simulink model "quadrotor_1d"  (R2025b)
settings: Solver=VariableStepAuto  StartTime=0.0  StopTime=20  RelTol=1e-3
values from neighbouring files (symbols this model uses):
  c_d = 0.1    [quad_params.m]
  g = 9.81    [quad_params.m]
  k_f = m*g/(4*w_hover^2)    (= 5.00510204082e-06)    [quad_params.m]
  Kd = m*(2*zeta*wn + alpha)    [design_pid.m]
  Ki = m*(alpha*wn^2)    [design_pid.m]
  Kp = m*(wn^2 + 2*zeta*wn*alpha)    [design_pid.m]
  m = 1.0    (= 1)    [quad_params.m]
  tau_m = 0.05    [quad_params.m]
  U_max = 2*m*g    (= 19.62)    [quad_params.m]
  w_hover = 700    [quad_params.m]
  w_max = sqrt(U_max/(4*k_f))    [quad_params.m]
  wind_amp = -6    [quad_params.m]
  wind_dur = 3    [quad_params.m]
  wind_t0 = 5    [quad_params.m]
  z0 = 0    [quad_params.m]
settings Model: Creator=Monster  LastModifiedBy=Monster

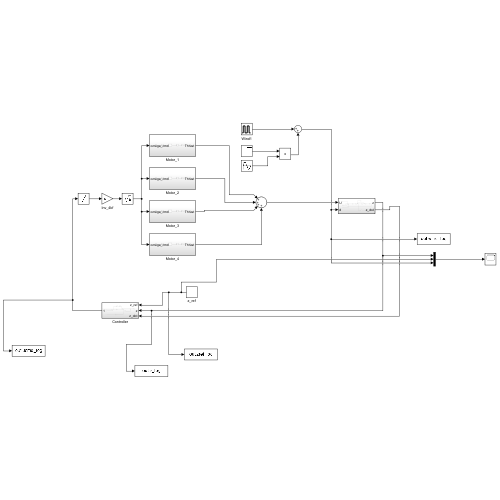
[thumbnail: Simulink's stored preview of the top-level diagram]
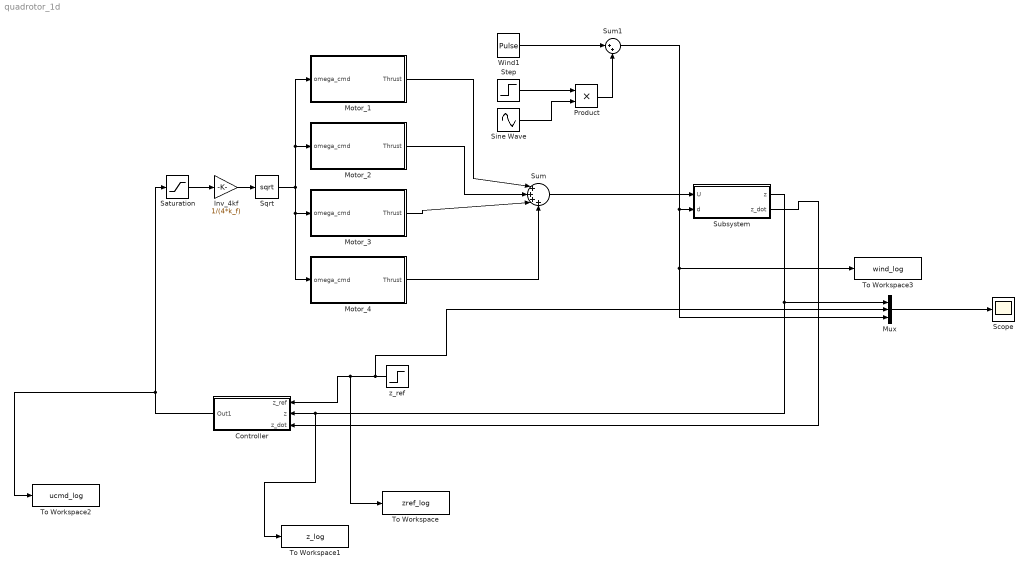
== system quadrotor_1d ==
  Controller : Subsystem
  Inv_4kf : Gain  Gain=1/(4*k_f)
  Motor_1 : Subsystem
  Motor_2 : Subsystem
  Motor_3 : Subsystem
  Motor_4 : Subsystem
  Mux : Mux  Inputs=3
  Product : Product
  Saturation : Saturate  UpperLimit=U_max  LowerLimit=0
  Scope : Scope
      settings: ActiveDisplayYMinimum=-11.330608642093068  ActiveDisplayYMaximum=2.393195803335681
  Sine Wave : Sin  Amplitude=3  Frequency=2  Phase=-24  SampleTime=0
  Sqrt : Sqrt
  Step : Step  Time=12  SampleTime=0
  Subsystem : Subsystem
  Sum : Sum  Inputs=|++++
  Sum1 : Sum  Inputs=|++
  To Workspace : ToWorkspace  VariableName=zref_log  SampleTime=-1
  To Workspace1 : ToWorkspace  VariableName=z_log  SampleTime=-1
  To Workspace2 : ToWorkspace  VariableName=ucmd_log  SampleTime=-1
  To Workspace3 : ToWorkspace  VariableName=wind_log  SampleTime=-1
  Wind1 : DiscretePulseGenerator  PulseType=Time based  Amplitude=wind_amp  Period=20  PulseWidth=100*wind_dur/20  PhaseDelay=wind_t0
  z_ref : Step  After=0.2  SampleTime=0
  wires:
  Inv_4kf/1 -> Sqrt/1
  Controller/1(Out1) -> To Workspace2/1, Saturation/1
  Saturation/1 -> Inv_4kf/1
  Sqrt/1 -> Motor_2/1(omega_cmd), Motor_1/1(omega_cmd), Motor_4/1(omega_cmd), Motor_3/1(omega_cmd)
  Motor_1/1(Thrust) -> Sum/1
  Motor_2/1(Thrust) -> Sum/2
  Motor_3/1(Thrust) -> Sum/3
  Motor_4/1(Thrust) -> Sum/4
  Sum/1 -> Subsystem/1(U)
  Sum1/1 -> Mux/3, To Workspace3/1, Subsystem/2(d)
  Subsystem/2(z_dot) -> Controller/3(z_dot)
  Subsystem/1(z) -> To Workspace1/1, Controller/2(z), Mux/1
  Mux/1 -> Scope/1
  z_ref/1 -> Mux/2, To Workspace/1, Controller/1(z_ref)
  Sine Wave/1 -> Product/2
  Step/1 -> Product/1
  Wind1/1 -> Sum1/1
  Product/1 -> Sum1/2

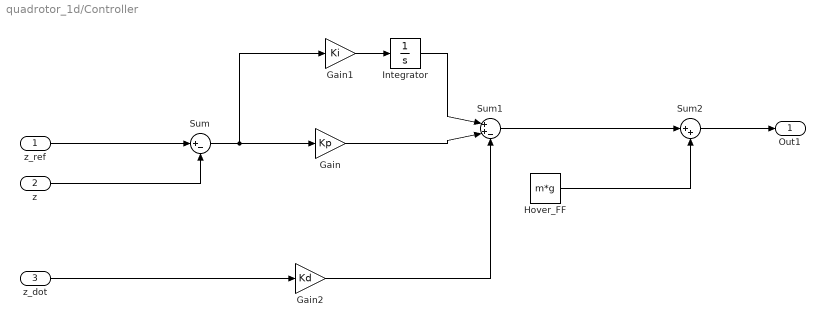
== system quadrotor_1d/Controller ==
  z_ref : Inport
  z : Inport  Port=2
  z_dot : Inport  Port=3
  Gain : Gain  Gain=Kp
  Gain1 : Gain  Gain=Ki
  Gain2 : Gain  Gain=Kd
  Hover_FF : Constant  Value=m*g
  Integrator : Integrator
  Sum : Sum  Inputs=|+-
  Sum1 : Sum  Inputs=|++-
  Sum2 : Sum  Inputs=|++
  Out1 : Outport
  wires:
  z_ref/1 -> Sum/1
  z/1 -> Sum/2
  Sum/1 -> Gain1/1, Gain/1
  Gain1/1 -> Integrator/1
  Integrator/1 -> Sum1/1
  Gain/1 -> Sum1/2
  z_dot/1 -> Gain2/1
  Gain2/1 -> Sum1/3
  Sum1/1 -> Sum2/1
  Hover_FF/1 -> Sum2/2
  Sum2/1 -> Out1/1

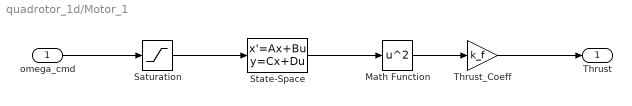
== system quadrotor_1d/Motor_1 ==
  omega_cmd : Inport
  Math Function : Math  Operator=square
  Saturation : Saturate  UpperLimit=w_max  LowerLimit=0
  State-Space : StateSpace  A=-1/tau_m  B=1/tau_m  D=0  InitialCondition=w_hover
  Thrust_Coeff : Gain  Gain=k_f
  Thrust : Outport
  wires:
  Thrust_Coeff/1 -> Thrust/1
  Saturation/1 -> State-Space/1
  State-Space/1 -> Math Function/1
  Math Function/1 -> Thrust_Coeff/1
  omega_cmd/1 -> Saturation/1

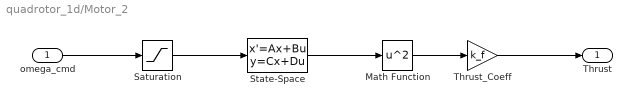
== system quadrotor_1d/Motor_2 ==
  omega_cmd : Inport
  Math Function : Math  Operator=square
  Saturation : Saturate  UpperLimit=w_max  LowerLimit=0
  State-Space : StateSpace  A=-1/tau_m  B=1/tau_m  D=0  InitialCondition=w_hover
  Thrust_Coeff : Gain  Gain=k_f
  Thrust : Outport
  wires:
  Thrust_Coeff/1 -> Thrust/1
  Saturation/1 -> State-Space/1
  State-Space/1 -> Math Function/1
  Math Function/1 -> Thrust_Coeff/1
  omega_cmd/1 -> Saturation/1

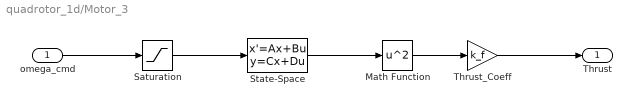
== system quadrotor_1d/Motor_3 ==
  omega_cmd : Inport
  Math Function : Math  Operator=square
  Saturation : Saturate  UpperLimit=w_max  LowerLimit=0
  State-Space : StateSpace  A=-1/tau_m  B=1/tau_m  D=0  InitialCondition=w_hover
  Thrust_Coeff : Gain  Gain=k_f
  Thrust : Outport
  wires:
  Thrust_Coeff/1 -> Thrust/1
  Saturation/1 -> State-Space/1
  State-Space/1 -> Math Function/1
  Math Function/1 -> Thrust_Coeff/1
  omega_cmd/1 -> Saturation/1

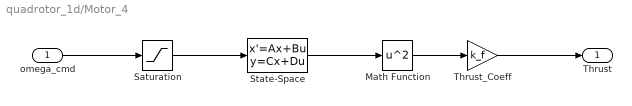
== system quadrotor_1d/Motor_4 ==
  omega_cmd : Inport
  Math Function : Math  Operator=square
  Saturation : Saturate  UpperLimit=w_max  LowerLimit=0
  State-Space : StateSpace  A=-1/tau_m  B=1/tau_m  D=0  InitialCondition=w_hover
  Thrust_Coeff : Gain  Gain=k_f
  Thrust : Outport
  wires:
  Thrust_Coeff/1 -> Thrust/1
  Saturation/1 -> State-Space/1
  State-Space/1 -> Math Function/1
  Math Function/1 -> Thrust_Coeff/1
  omega_cmd/1 -> Saturation/1

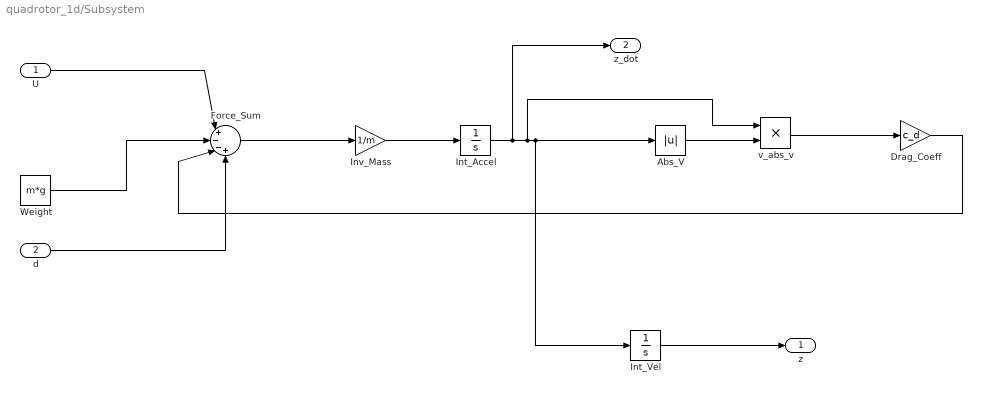
== system quadrotor_1d/Subsystem ==
  U : Inport
  d : Inport  Port=2
  Abs_V : Abs  SaturateOnIntegerOverflow=off
  Drag_Coeff : Gain  Gain=c_d
  Force_Sum : Sum  Inputs=|+--+
  Int_Accel : Integrator
  Int_Vel : Integrator  InitialCondition=z0
  Inv_Mass : Gain  Gain=1/m
  Weight : Constant  Value=m*g
  v_abs_v : Product
  z : Outport
  z_dot : Outport  Port=2
  wires:
  U/1 -> Force_Sum/1
  Weight/1 -> Force_Sum/2
  d/1 -> Force_Sum/4
  Drag_Coeff/1 -> Force_Sum/3
  Force_Sum/1 -> Inv_Mass/1
  Inv_Mass/1 -> Int_Accel/1
  Int_Accel/1 -> z_dot/1, v_abs_v/1, Abs_V/1, Int_Vel/1
  Abs_V/1 -> v_abs_v/2
  v_abs_v/1 -> Drag_Coeff/1
  Int_Vel/1 -> z/1
